simulink model "p88_stop_sign_detector"  (R2026a)
settings: Solver=ode3  StopTime=inf  EnableMultiTasking=on
StopFcn:
  | h=findobj('type','figure');if ~isempty(h);close(h); clear h; end
model workspace (MAT data in the model file):
  RGB_image = [255 255 255 255 255 255 255 255 255 255 255 255 ... (230400 elements, 240x320x3)]
libraries: raspberrypiAVlib x2
(part 2 of 2)

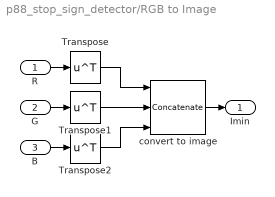
== system p88_stop_sign_detector/RGB to Image ==
  R : Inport
  G : Inport  Port=2
  B : Inport  Port=3
  Transpose : Math  Operator=transpose
  Transpose1 : Math  Operator=transpose
  Transpose2 : Math  Operator=transpose
  convert to image : Concatenate  NumInputs=3  Mode=Multidimensional array  ConcatenateDimension=3
  Imin : Outport
  wires:
  R/1 -> Transpose/1
  G/1 -> Transpose1/1
  Transpose/1 -> convert to image/1
  Transpose1/1 -> convert to image/2
  B/1 -> Transpose2/1
  Transpose2/1 -> convert to image/3
  convert to image/1 -> Imin/1

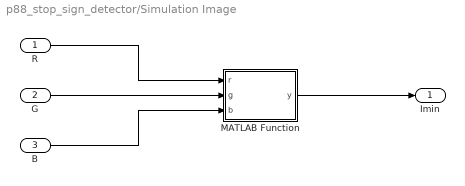
== system p88_stop_sign_detector/Simulation Image ==
  R : Inport
  G : Inport  Port=2
  B : Inport  Port=3
  MATLAB Function : MATLAB Function  TreatAsAtomicUnit=on
  Imin : Outport
  wires:
  G/1 -> MATLAB Function/2(g)
  R/1 -> MATLAB Function/1(r)
  B/1 -> MATLAB Function/3(b)
  MATLAB Function/1(y) -> Imin/1

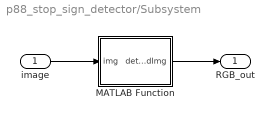
== system p88_stop_sign_detector/Subsystem ==
  image : Inport
  MATLAB Function : MATLAB Function  TreatAsAtomicUnit=on
  RGB_out : Outport
  wires:
  image/1 -> MATLAB Function/1(img)
  MATLAB Function/1(detectedImg) -> RGB_out/1

== matlab function p88_stop_sign_detector/Subsystem/MATLAB Function ==
  data: img input; detectedImg output
function detectedImg = fcn(img)
%#codegen

persistent detector

% 최초 실행 때 학습된 검출기 불러오기
if isempty(detector)
    detector = vision.CascadeObjectDetector('/sdcard/stop_sign_detector/stopSignDetector.xml');
end

% 입력 이미지에서 STOP 표지판 위치 찾기
bbox = step(detector, img);

% 검출 위치에 사각형과 글자 표시
detectedImg = insertObjectAnnotation( ...
    img, 'rectangle', bbox, 'stop sign');

end

== matlab function p88_stop_sign_detector/MATLAB Function ==
  data: RGB_out input
function image_display(RGB_out)
% image_display is MatLAB function block created to automatically display
% an RGB channel stream as an image using imshow matlab command
%
% See also 'imshow'

% Declaration to use 'imshow' with coder.extrinsic
coder.extrinsic('imshow');
% persistent hFig; % Figure variable and reusing it for display
% if isempty(hFig)
%     hFig = figure('Position',[0 0 1024 768]);
% end
imshow(RGB_out); % Display image in figure
end

== matlab function p88_stop_sign_detector/ImageToRGB ==
  data: i input; R output; G output; B output
function [R,G,B] = ImageToRGB(i)
%#codegen
R =i(:,:,1)';
G =i(:,:,2)';
B =i(:,:,3)';
end

== matlab function p88_stop_sign_detector/Simulation Image/MATLAB Function ==
  data: r input; y output; g input; b input
function y = fcn(r, g, b)
%#codegen

% R, G, B를 하나의 RGB 이미지로 합치기
y = cat(3, r, g, b);

end
